simulink model "Simulink_08"  (R2025b)
settings: Solver=ode45  StartTime=0.0  StopTime=10  RelTol=1e-3
settings Model: Creator=Nico6700  LastModifiedBy=Nico6700

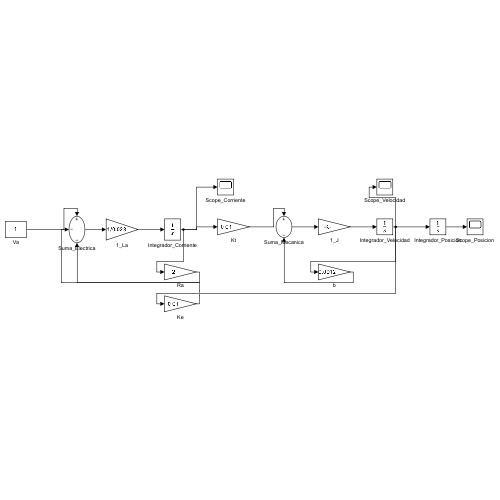
[thumbnail: Simulink's stored preview of the top-level diagram]
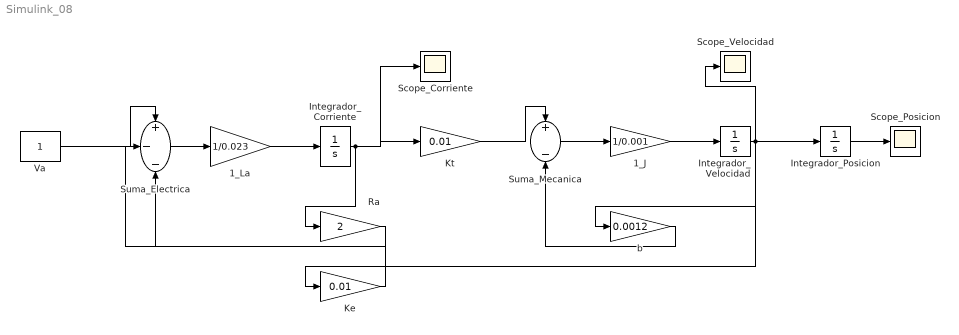
== system Simulink_08 ==
  1_J : Gain  Gain=1/0.001
  1_La : Gain  Gain=1/0.023
  Integrador_Corriente : Integrator
  Integrador_Posicion : Integrator
  Integrador_Velocidad : Integrator
  Ke : Gain  Gain=0.01
  Kt : Gain  Gain=0.01
  Ra : Gain  Gain=2
  Scope_Corriente : Scope
      settings: ActiveDisplayYMinimum=-0.062270632804103221  ActiveDisplayYMaximum=0.56043569523692915
  Scope_Posicion : Scope
      settings: ActiveDisplayYMinimum=-4.594481496022718  ActiveDisplayYMaximum=41.350333464204468
  Scope_Velocidad : Scope
      settings: ActiveDisplayYMinimum=-0.50000494729003631  ActiveDisplayYMaximum=4.5000445256103276
  Suma_Electrica : Sum  Inputs=+--
  Suma_Mecanica : Sum  Inputs=+-
  Va : Constant
  b : Gain  Gain=0.0012
  wires:
  Va/1 -> Suma_Electrica/1
  Suma_Electrica/1 -> 1_La/1
  1_La/1 -> Integrador_Corriente/1
  Integrador_Corriente/1 -> Ra/1, Kt/1, Scope_Corriente/1
  Ra/1 -> Suma_Electrica/2
  Kt/1 -> Suma_Mecanica/1
  Suma_Mecanica/1 -> 1_J/1
  1_J/1 -> Integrador_Velocidad/1
  Integrador_Velocidad/1 -> b/1, Ke/1, Scope_Velocidad/1, Integrador_Posicion/1
  b/1 -> Suma_Mecanica/2
  Ke/1 -> Suma_Electrica/3
  Integrador_Posicion/1 -> Scope_Posicion/1
